simulink model "cp5_ej1"  (R2026a)
settings: Solver=VariableStepAuto  StopTime=20  MaxStep=0.01
settings Model: Creator=benja  LastModifiedBy=benja

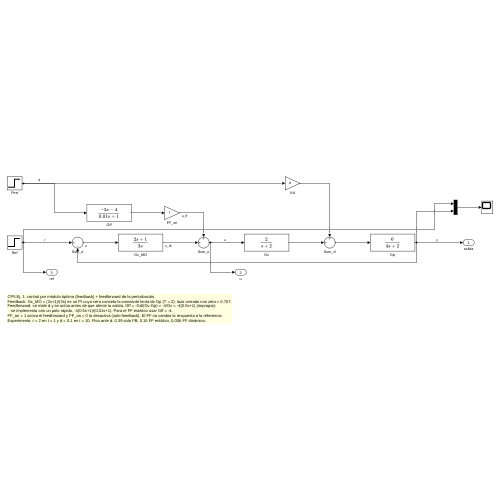
[thumbnail: Simulink's stored preview of the top-level diagram]
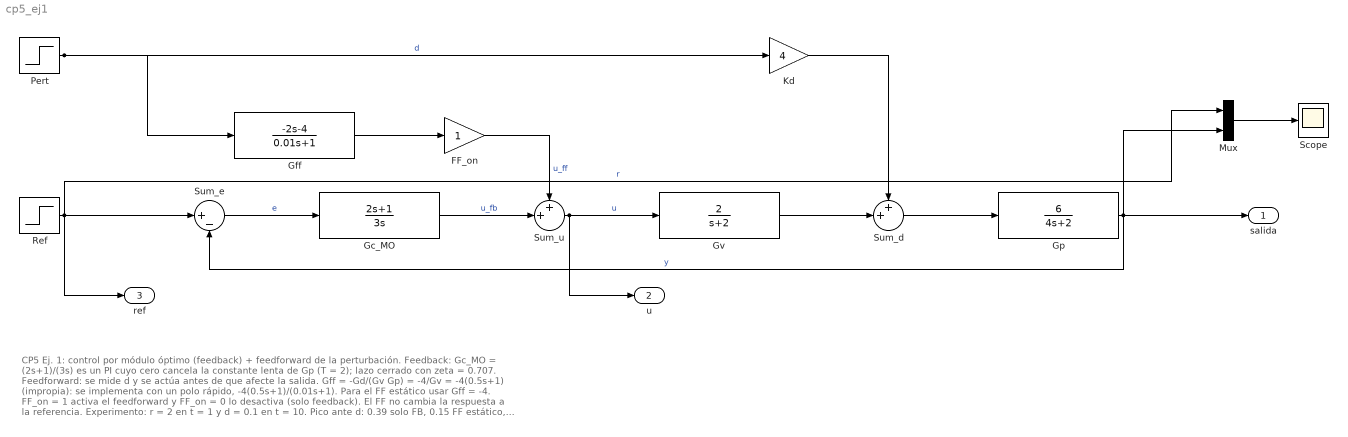
== system cp5_ej1 ==
  note: CP5 Ej. 1: control por módulo óptimo (feedback) + feedforward de la perturbación.
      | Feedback: Gc_MO = (2s+1)/(3s) es un PI cuyo cero cancela la constante lenta de Gp (T = 2); lazo cerrado con zeta = 0.707.
      | Feedforward: se mide d y se actúa antes de que afecte la salida. Gff = -Gd/(Gv Gp) = -4/Gv = -4(0.5s+1) (impropia):
      |    se implementa con un polo rápido, -4(0.5s+1)/(0.01s+1). Para el FF estático usar Gff = -4.
      | FF_on = 1 activa el feedforward y FF_on = 0 lo desactiva (solo feedback). El FF no cambia la respuesta a la referencia.
      | Experimento: r = 2 en t = 1 y d = 0.1 en t = 10. Pico ante d: 0.39 solo FB, 0.15 FF estático, 0.006 FF dinámico.
  FF_on : Gain
  Gc_MO : TransferFcn  Numerator=[2 1]  Denominator=[3 0]
  Gff : TransferFcn  Numerator=[-2 -4]  Denominator=[0.01 1]
  Gp : TransferFcn  Numerator=6  Denominator=[4 2]
  Gv : TransferFcn  Numerator=2  Denominator=[1 2]
  Kd : Gain  Gain=4
  Mux : Mux  Inputs=2
  Pert : Step  Time=10  FinalValue=0.1  SampleTime=0
  Ref : Step  FinalValue=2  SampleTime=0
  Scope : Scope
  Sum_d : Sum  Inputs=++|
  Sum_e : Sum  Inputs=|+-
  Sum_u : Sum  Inputs=++|
  salida : Outport
  u : Outport  Port=2
  ref : Outport  Port=3
  wires:
  Ref/1 -> Sum_e/1, ref/1, Mux/1  "r"
  Sum_e/1 -> Gc_MO/1  "e"
  Gc_MO/1 -> Sum_u/2  "u_fb"
  Pert/1 -> Gff/1, Kd/1  "d"
  Gff/1 -> FF_on/1
  FF_on/1 -> Sum_u/1  "u_ff"
  Sum_u/1 -> Gv/1, u/1  "u"
  Gv/1 -> Sum_d/2
  Kd/1 -> Sum_d/1
  Sum_d/1 -> Gp/1
  Gp/1 -> salida/1, Sum_e/2, Mux/2  "y"
  Mux/1 -> Scope/1
